simulink model "mrsDiffDriveWaypointLogicModelDEMO"  (R2026a)
settings: Solver=VariableStepAuto  StopTime=140  FixedStep=0.01  EnableMultiTasking=on
PreLoadFcn:
  | % Simulation parameters
  | sampleTime = 0.05;
  | 
  | % Vehicle parameters
  | R = 0.1;
  | L = 0.5;
libraries: mobileRoboticsLib x3
settings Model: Creator=scastro  LastModifiedBy=merwinmendoza
settings DebuggingCC: PregeneratedLibrarySubsystemCodeDiagnostic=none
settings SimscapeCC: SimscapeNominalValues="[{\"value\":\"10\",\"unit\":\"V\"},{\"value\":\"1\",\"unit\":\"A\"},{\"value\":\"10\",\"unit\":\"N*m\"},{\"value\":\"10\",\"unit\":\"bar\"},{\"value\":\"100\",\"unit\":\"kJ/kg\"},{\"value\":\"1\",\"unit\":\"kW\"},{\"value\":\"300\",\"unit\":\"K\"},{\"value\":\"100\",\"unit\":\"cm^3/s\"},{\"value\":\"1\",\"unit\":\"kN\"},{\"value\":\"1\",\"unit\":\"g/cm^3\"},{\"value\":\"1\",\"unit\":\"l\"},{\"value\":\"1\",\"unit\":\"cm^2\"},{\"value\":\"60\",\"unit\":\"Hz\"}]"
settings ConfigurationSet: Description=SimMechanics 2G
settings ExplorerConfigSet: InternalSimMechanicsExplorerSettings="<ExplorerConfiguration><canonicalview>default</canonicalview><AnimationSetting><BasePlaybackSpeed>1.0</BasePlaybackSpeed><PlaybackSpeedFactor>1.0</PlaybackSpeedFactor></AnimationSetting><TilePanel><TileInfo><Tiles Columns=\"1\" Count=\"1\" Rows=\"1\"><Column Weight=\"1\"/><Row Weight=\"1\"/><Tile Height=\"1\" Width=\"1\" X=\"0\" Y=\"0\"/></Tiles></TileInfo><SceneInfo><SceneViewer><BGColor><R>0.60000002384185791</R><G>0.60000002384185791</G><B>0.60000002384185791</B></BGColor><Camera><DoPerspective>off</DoPerspective><Position><X>-1.70656042355848525</X><Y>-0.974920623359631922</Y><Z>4.72930454537082046</Z></Position><Center><X>0.552860638431633689</X><Y>1.42025063411503494</Y><Z>1.4843509506914252</Z></Center><Up><X>0.664249622453917166</X><Y>0.300615402055903091</Y><Z>0.684399604848363485</Z></Up><ViewLimDist>1</ViewLimDist><YLim>2.77881717169207398</YLim><XLim>3.55928742670435394</XLim></Camera></SceneViewer></SceneInfo></TilePanel><MechEditorPanel><Cameras/><GfxPanelCameraMap/><VideoCreator><PlaybackSpeedRatio>1.0</PlaybackSpeedRatio><FrameRate>30</FrameRate><VideoFormat>Motion JPEG AVI</VideoFormat><FrameSize>auto</FrameSize></VideoCreator></MechEditorPanel></ExplorerConfiguration>"

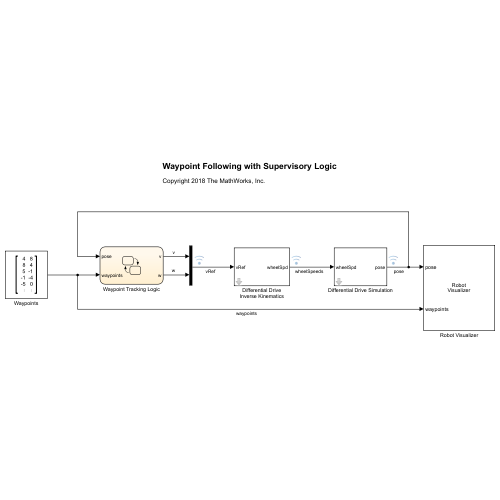
[thumbnail: Simulink's stored preview of the top-level diagram]
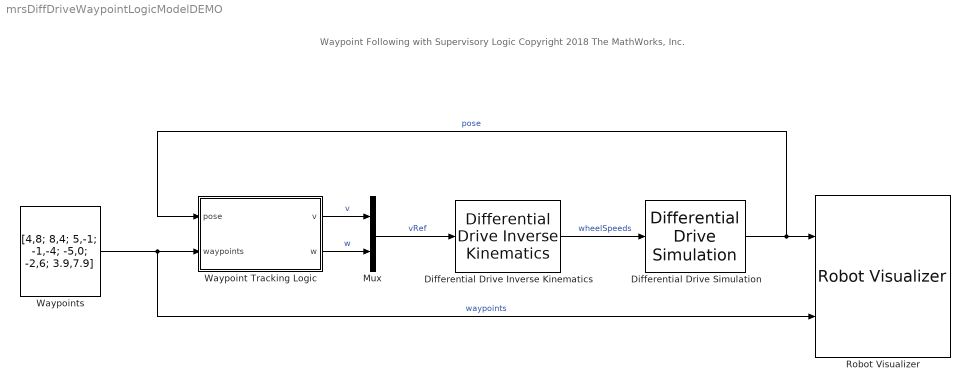
== system mrsDiffDriveWaypointLogicModelDEMO ==
  note: Waypoint Following with Supervisory Logic
      |
      | Copyright 2018 The MathWorks, Inc.
  Differential Drive Inverse Kinematics : mobileRoboticsLib/Kinematic Models/Differential Drive/Differential Drive Inverse Kinematics  wheelRadius=R  wheelBase=L
      settings: SourceProductName=Mobile Robotics Simulation Toolbox
  Differential Drive Simulation : mobileRoboticsLib/Kinematic Models/Differential Drive/Differential Drive Simulation  wheelRadius=R  wheelBase=L  initX=0  initY=0  initAngle=0  Ts=sampleTime
      settings: SourceProductName=Mobile Robotics Simulation Toolbox
  Mux : Mux  Inputs=2
  Robot Visualizer : mobileRoboticsLib/Environments/Robot Visualizer  Priority=99  robotRadius=0  showTrajectory=on  hasWaypoints=on  hasLidar=off  sensorOffset=[ 0 0 ]  scanAngles=0  hasObjDetector=off  objDetectorOffset=[ 0, 0 ]  objDetectorAngle=0  objDetectorFOV=0  objDetectorMaxRange=0  objectColors=0  objectMarkers=s
  Waypoint Tracking Logic : Stateflow chart  TreatAsAtomicUnit=on
  Waypoints : Constant  Value=[4,8; 8,4; 5,-1; -1,-4; -5,0; -2,6; 3.9,7.9]
  wires:
  Differential Drive Simulation/1 -> Waypoint Tracking Logic/1(pose), Robot Visualizer/1  "pose"
  Differential Drive Inverse Kinematics/1 -> Differential Drive Simulation/1  "wheelSpeeds"
  Waypoint Tracking Logic/2(w) -> Mux/2  "w"
  Mux/1 -> Differential Drive Inverse Kinematics/1  "vRef"
  Waypoint Tracking Logic/1(v) -> Mux/1  "v"
  Waypoints/1 -> Robot Visualizer/2, Waypoint Tracking Logic/2(waypoints)  "waypoints"

== stateflow chart mrsDiffDriveWaypointLogicModelDEMO/Waypoint Tracking Logic ==
  state FollowWaypoints
    entry:
    goalPoint = waypoints(idx,:);
    entry, during:
    [angle,range] = trackGoal(goalPoint);
    (default) -> (junction 20)
    FollowWaypoints -> (junction 20) [order 1]
    (junction 20) -> (junction 24) [order 1] : % Set angular speed if
        | % angle outside deadband
        | [abs(angle) > pi/24]
    (junction 20) -> (junction 30) [order 2] : {w = 0;}
    (junction 24) -> (junction 49) : % Proportional
        | % control
        | {w = 1.5*angle;}
    (junction 49) -> (junction 30)
  state ReachedGoal
    entry:
    v = 0;
    w = 0.5;
  (default) -> FollowWaypoints : {
      | v = 0.5;
      | idx = 1;
      | numPts = size(waypoints,1);
      | }
  FollowWaypoints -> (junction 39) [order 1] : % Check if goal reached
      | [range < 0.1]
  (junction 39) -> ReachedGoal [order 1] : % Stop if final waypoint
      | [idx == numPts]
  (junction 39) -> (junction 42) [order 2]
  (junction 42) -> FollowWaypoints : % Go to the next waypoint
      | {idx = idx + 1;}
  data: goal function_input; ang function_output; dist function_output; pose input; waypoints input; v output; w output; angle local; range local; idx local; numPts local; goalPoint local
  function [ang,dist] = trackGoal(goal):
    | function [ang,dist] = trackGoal(goal)
    | % Finds the angle (theta) and distance (dist) between the 
    | % vehicle and a goal point
    |     
    | posDiff = [goal(1)-pose(1);goal(2)-pose(2)];
    | 
    | ang = angdiff(pose(3),atan2(posDiff(2),posDiff(1)));
    | dist = sqrt(posDiff(1)^2 + posDiff(2)^2);
